simulink model "UAV_GuidanceStepResponse"  (R2026a)
settings: Solver=ode45  StopTime=10  MaxStep=0.01
model workspace (MAT data in the model file):
  dPitch = 0
  dRoll = 0
  dThrust = 0
  dYawRate = 0
  gravityNED = 9.81
  hoverThrust = 0.981
  tStep = 1
  uavMass = 0.1
libraries: uavalgslib x1
settings Model: Creator=PattarapolSangaroon  LastModifiedBy=PattarapolSangaroon

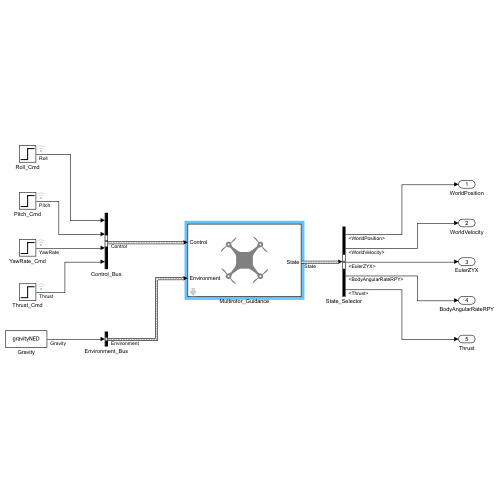
[thumbnail: Simulink's stored preview of the top-level diagram]
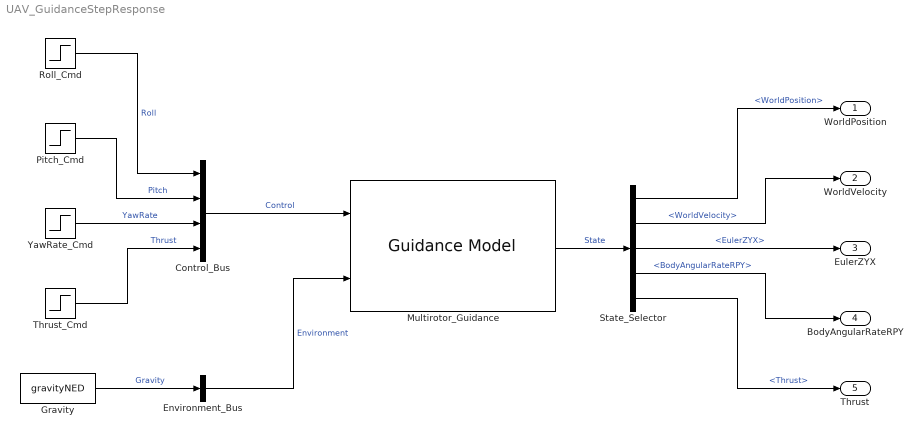
== system UAV_GuidanceStepResponse ==
  Control_Bus : BusCreator  Inputs=4  OutDataTypeStr=Bus: MultirotorGuidanceControlBus  NonVirtualBus=on
  Environment_Bus : BusCreator  Inputs=1  OutDataTypeStr=Bus: MultirotorGuidanceEnvironmentBus  NonVirtualBus=on
  Gravity : Constant  Value=gravityNED
  Multirotor_Guidance : uavalgslib/Guidance Model  ModelType=MultirotorGuidance  NumInstances=1  SpecifiedDataType=double  SimulateUsing=Interpreted execution  InitialWorldPositionMultirotor=[0; 0; 0]  InitialWorldVelocityMultirotor=[0; 0; 0]  InitialEulerZYXMultirotor=[0; 0; 0]  InitialBodyAngularRateRPYMultirotor=[0; 0; 0]  InitialThrustMultirotor=hoverThrust  InitialNorthFixedWing=0  InitialEastFixedWing=0  InitialHeightFixedWing=0  InitialAirSpeedFixedWing=0  InitialHeadingAngleFixedWing=0  InitialFlightPathAngleFixedWing=0  InitialRollAngleFixedWing=0  InitialRollAngleRateFixedWing=0  PDRollMultirotor=[3402.97,116.67]  PDPitchMultirotor=[3402.97, 116.67]  PYawRateMultirotor=1950  PThrustMultirotor=3900  MassMultirotor=uavMass  PHeightFixedWing=3.9  PHeadingAngleFixedWing=3.9  PFlightPathAngleFixedWing=39  PDRollFixedWing=[3402.97, 116.67]  PAirSpeedFixedWing=1  FlightPathAngleLimitsFixedWing=[-pi/2, pi/2]  StateBusName='MultirotorGuidanceStateBus'  ControlBusName='MultirotorGuidanceControlBus'  EnvironmentBusName='MultirotorGuidanceEnvironmentBus'  DataType=double
  Pitch_Cmd : Step  Time=tStep  FinalValue=dPitch  SampleTime=0
  Roll_Cmd : Step  Time=tStep  FinalValue=dRoll  SampleTime=0
  State_Selector : BusSelector  OutputSignals=WorldPosition,WorldVelocity,EulerZYX,BodyAngularRateRPY,Thrust
  Thrust_Cmd : Step  Time=tStep  InitialValue=hoverThrust  FinalValue=hoverThrust + dThrust  SampleTime=0
  YawRate_Cmd : Step  Time=tStep  FinalValue=dYawRate  SampleTime=0
  WorldPosition : Outport
  WorldVelocity : Outport  Port=2
  EulerZYX : Outport  Port=3
  BodyAngularRateRPY : Outport  Port=4
  Thrust : Outport  Port=5
  wires:
  Multirotor_Guidance/1 -> State_Selector/1  "State"
  Environment_Bus/1 -> Multirotor_Guidance/2  "Environment"
  Control_Bus/1 -> Multirotor_Guidance/1  "Control"
  Roll_Cmd/1 -> Control_Bus/1  "Roll"
  Pitch_Cmd/1 -> Control_Bus/2  "Pitch"
  YawRate_Cmd/1 -> Control_Bus/3  "YawRate"
  Thrust_Cmd/1 -> Control_Bus/4  "Thrust"
  Gravity/1 -> Environment_Bus/1  "Gravity"
  State_Selector/1 -> WorldPosition/1  "<WorldPosition>"
  State_Selector/2 -> WorldVelocity/1  "<WorldVelocity>"
  State_Selector/3 -> EulerZYX/1  "<EulerZYX>"
  State_Selector/4 -> BodyAngularRateRPY/1  "<BodyAngularRateRPY>"
  State_Selector/5 -> Thrust/1  "<Thrust>"
